simulink model "flex_slew"  (R2025b)
settings: Solver=ode45  StartTime=0.0  StopTime=t_out(end)  RelTol=1e-10  AbsTol=1e-12
model workspace (MAT data in the model file):
  A = [0  0  0  0  0  0  0  1  0  0  0  0  0  0; 0  0  0  0  0  0  0  0  1  0  0  0  0  0; 0  0  0  0  0  0  0  0  0  1  0  0  0  0; 0  0  0  0  0  0  0  0  0  0  1  0  0  0; 0  0  0  0  0  0  0  0  0  0  0  1  0  0; 0  0  0  0  0  0  0  0  0  0  0  0  1  0; 0  0  0  0  0  0  0  0  0  0  0  0  0  1; 0  0.215391156389  1.97278428303  7.09577677888  0.215391156389  1.97278428303  7.09577677888  0  0.000857014180941  0.00125252804303  0.00160896012531  0.000857014180941  0.00125252804303  0.00160896012531; 0  -7.42343413162  -10.1380666438  -36.464938662  -1.10688731492  -10.1380666438  -36.464938662  0  -0.0295369059191  -0.00643669603552  -0.00826838753631  -0.00440416469039  -0.00643669603552  -0.00826838753631; 0  -0.258137190412  -250.440030979  -8.50398833545  -0.258137190412  -2.36429851925  -8.50398833545  0  -0.00102709524625  -0.159005302605  -0.0019282706551  -0.00102709524625  -0.00150110188069  -0.0019282706551; 0  -0.118425677871  -1.08466995547  -1948.85534651  -0.118425677871  -1.08466995547  -3.90137733203  0  -0.000471200800553  -0.000688660969348  -0.441900956052  -0.000471200800553  -0.000688660969348  -0.000884633318751; 0  -1.10688731492  -10.1380666438  -36.464938662  -7.42343413162  -10.1380666438  -36.464938662  0  -0.00440416469039  -0.00643669603552  -0.00826838753631  -0.0295369059191  -0.00643669603552  -0.00826838753631; 0  -0.258137190412  -2.36429851925  -8.50398833545  -0.258137190412  -250.440030979  -8.50398833545  0  -0.00102709524625  -0.00150110188069  -0.0019282706551  -0.00102709524625  -0.159005302605  -0.0019282706551; 0  -0.118425677871  -1.08466995547  -3.90137733203  -0.118425677871  -1.08466995547  -1948.85534651  0  -0.000471200800553  -0.000688660969348  -0.000884633318751  -0.000471200800553  -0.000688660969348  -0.441900956052]
  Ak = [9.80954112128  -2.47347256621  0  0; 76.8214220921  22.4350675726  39.5716474757  0; 0  -33.5608178632  -32.0425440976  -64.4448608345; 0  0  2.86857600503  -11.4060178503]
  B = [0; 0; 0; 0; 0; 0; 0; 0.00663548399581; -0.0340995107991; -0.0079523469042; -0.00364830062374; -0.0340995107991; -0.0079523469042; -0.00364830062374]
  Bk = [92.2546966114  43.3313842252; 91.3564986664  232.256698891; 0.220196740694  31.8382065476; 15.0156026314  96.1272142477]
  C = [1  0  0  0  0  0  0  0  0  0  0  0  0  0; 0  0  0  0  0  0  0  1  0  0  0  0  0  0; 0  0.816496580928  -0.816496580928  0.816496580928  0  0  0  0  0  0  0  0  0  0]
  Ck = [-111.898295617 -60.7037665154 -100.720832662 14.4931962202]
  D = [0; 0; 0]
  Dk = [5.56338197917 -734.876053796]
  J = 207
  Kd = 91.043355101
  Kp = 20.4300811103
  T = 40.3208903452
  a = 0.00386473429952
  t_out = [0 0.02 0.04 0.06 0.08 0.1 0.12 0.14 0.16 0.18 0.2 0.22 ... (6003 elements, 6003x1)]
  umax = 1
settings Model: Creator=avaza  LastModifiedBy=avaza
settings DataIOCC: SaveOutput=off  SaveTime=off  OutputOption=SpecifiedOutputTimes  OutputTimes=t_out

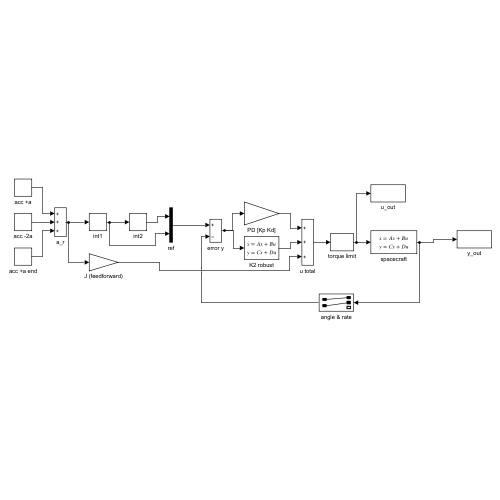
[thumbnail: Simulink's stored preview of the top-level diagram]
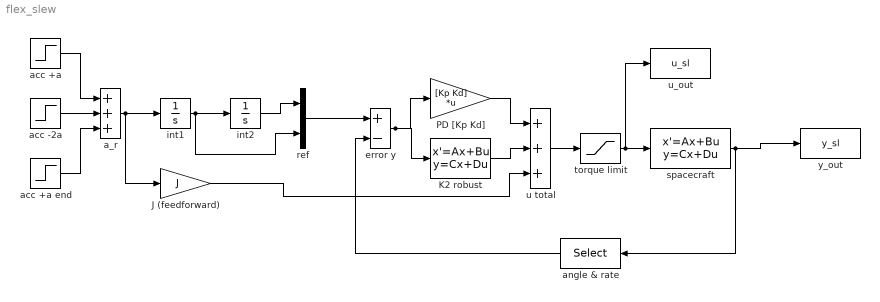
== system flex_slew ==
  J (feedforward) : Gain  Gain=J
  K2 robust : StateSpace  A=Ak  B=Bk  C=Ck  D=Dk  InitialCondition=0
  PD [Kp Kd] : Gain  Gain=[Kp Kd]  Multiplication=Matrix(K*u)
  a_r : Sum  Inputs=+++
  acc +a : Step  Time=0  After=a  SampleTime=0
  acc +a end : Step  Time=T  After=a  SampleTime=0
  acc -2a : Step  Time=T/2  After=-2*a  SampleTime=0
  angle & rate : Selector  InputPortWidth=3  IndexOptions=Index vector (dialog)  Indices=[1 2]  OutputSizes=1
  error y : Sum  Inputs=+-
  int1 : Integrator
  int2 : Integrator
  ref : Mux  Inputs=2
  spacecraft : StateSpace  A=A  B=B  C=C  D=D  InitialCondition=0
  torque limit : Saturate  UpperLimit=umax  LowerLimit=-umax
  u total : Sum  Inputs=+++
  u_out : ToWorkspace  VariableName=u_sl  SampleTime=-1
  y_out : ToWorkspace  VariableName=y_sl  SampleTime=-1
  wires:
  acc +a/1 -> a_r/1
  acc -2a/1 -> a_r/2
  acc +a end/1 -> a_r/3
  a_r/1 -> int1/1, J (feedforward)/1
  int1/1 -> int2/1, ref/2
  int2/1 -> ref/1
  ref/1 -> error y/1
  angle & rate/1 -> error y/2
  error y/1 -> PD [Kp Kd]/1, K2 robust/1
  PD [Kp Kd]/1 -> u total/1
  K2 robust/1 -> u total/2
  J (feedforward)/1 -> u total/3
  u total/1 -> torque limit/1
  torque limit/1 -> spacecraft/1, u_out/1
  spacecraft/1 -> y_out/1, angle & rate/1
